simulink model "servo_armature"  (R2023b)
settings: Solver=ode45  StartTime=0.0  StopTime=Tend  MaxStep=1e-3  RelTol=1e-8  AbsTol=1e-10
model workspace (MAT data in the model file):
  J = 1e-06
  Kd = 0
  Ke = 0.00568713663315
  Ki = 1
  KiOn = 1
  Kp = 0.05
  Kt = 0.00568713663315
  L = 0.0005
  N = 100
  R = 1.6
  Tend = 5
  Tf = 0.01
  Ts = 0.01
  aw = 1
  b = 2.41369575255e-06
  closedLoop = 1
  dist = 0
  eta = 1
  ffGain = 0.0666666666667
  loopSel = 1
  qInt = 0.0692307692308
  setpoint = 100
  tDist = 3
  tStep = 0.2
  uMax = 12
libraries: simulink x2
settings Model: Creator=odyssix  LastModifiedBy=odyssix
settings ModelReferenceCC: UpdateModelReferenceTargets=IfOutOfDate
settings RTWCC: GPUComputeCapability=5.0
settings ConfigComp: CovBoundaryAbsTol=1.0e-5

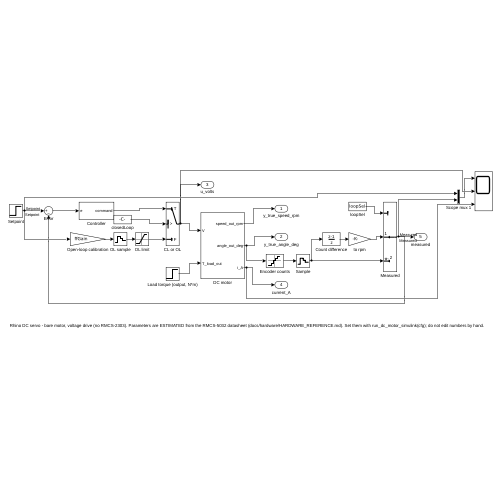
[thumbnail: Simulink's stored preview of the top-level diagram]
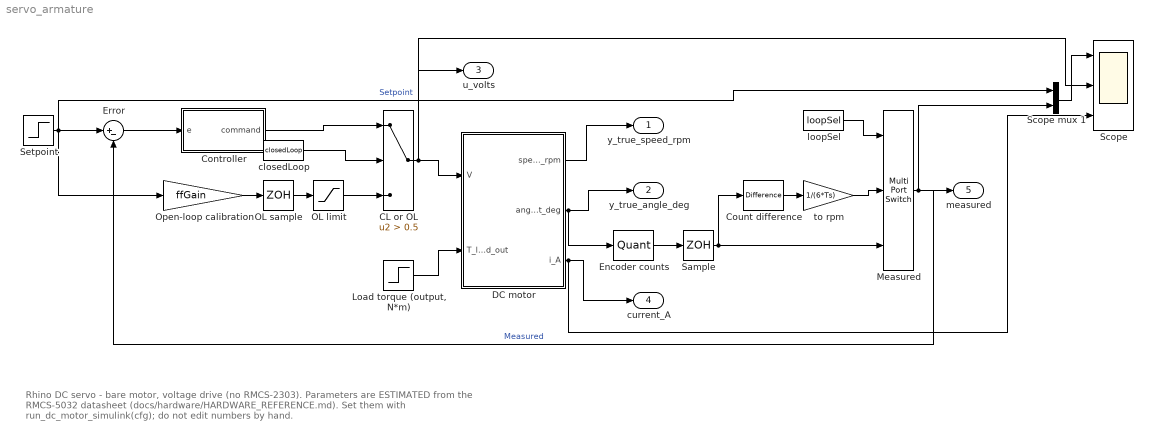
== system servo_armature ==
  note: Rhino DC servo - bare motor, voltage drive (no RMCS-2303). Parameters are ESTIMATED from the RMCS-5032 datasheet (docs/hardware/HARDWARE_REFERENCE.md). Set them with run_dc_motor_simulink(cfg); do not edit numbers by hand.
  CL or OL : Switch  Criteria=u2 > Threshold  Threshold=0.5  SaturateOnIntegerOverflow=off  InputSameDT=off
  Controller : Subsystem
  Count difference : simulink/Discrete/Difference  ICPrevInput=0.0  OutMin=[]  OutMax=[]  OutDataType=fixdt(1, 16)  OutScaling=2^-10  DoSatur=off
  DC motor : Subsystem
  Encoder counts : Quantizer  QuantizationInterval=qInt
  Error : Sum  Inputs=|+-
  "Load torque (output, N*m)" : Step  Time=tDist  After=dist  SampleTime=0
  Measured : MultiPortSwitch  Inputs=2  SaturateOnIntegerOverflow=off  InputSameDT=off
  OL limit : Saturate  UpperLimit=uMax  LowerLimit=-uMax
  OL sample : ZeroOrderHold  SampleTime=Ts
  Open-loop calibration : Gain  Gain=ffGain
  Sample : ZeroOrderHold  SampleTime=Ts
  Scope : Scope  NumInputPorts=3
  Scope mux 1 : Mux  Inputs=2
  Setpoint : Step  Time=tStep  After=setpoint  SampleTime=0
  closedLoop : Constant  Value=closedLoop
  loopSel : Constant  Value=loopSel
  to rpm : Gain  Gain=1/(6*Ts)
  y_true_speed_rpm : Outport
  y_true_angle_deg : Outport  Port=2
  u_volts : Outport  Port=3
  current_A : Outport  Port=4
  measured : Outport  Port=5
  wires:
  Setpoint/1 -> Error/1, Open-loop calibration/1, Scope mux 1/1  "Setpoint"
  Error/1 -> Controller/1(e)
  Controller/1(command) -> CL or OL/1
  closedLoop/1 -> CL or OL/2
  Open-loop calibration/1 -> OL sample/1
  OL sample/1 -> OL limit/1
  OL limit/1 -> CL or OL/3
  CL or OL/1 -> DC motor/1(V), u_volts/1, Scope/2
  "Load torque (output, N*m)"/1 -> DC motor/2(T_load_out)
  DC motor/1(speed_out_rpm) -> y_true_speed_rpm/1
  DC motor/2(angle_out_deg) -> y_true_angle_deg/1, Encoder counts/1
  DC motor/3(i_A) -> current_A/1, Scope/3
  Encoder counts/1 -> Sample/1
  Sample/1 -> Count difference/1, Measured/3
  Count difference/1 -> to rpm/1
  loopSel/1 -> Measured/1
  to rpm/1 -> Measured/2
  Measured/1 -> Error/2, measured/1, Scope mux 1/2  "Measured"
  Scope mux 1/1 -> Scope/1

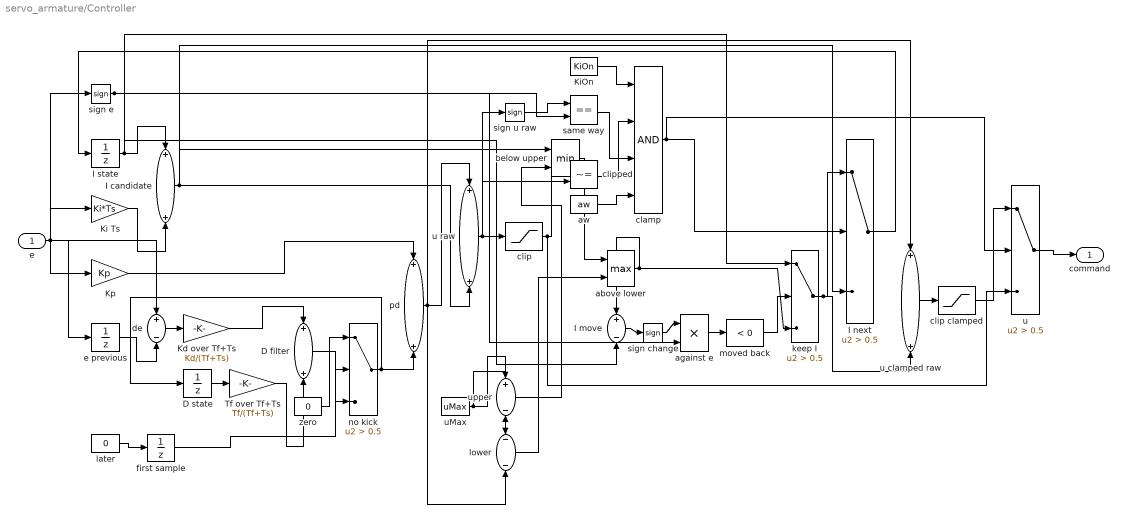
== system servo_armature/Controller ==
  e : Inport
  D filter : Sum
  D state : UnitDelay  SampleTime=Ts
  I candidate : Sum
  I move : Sum  Inputs=+-
  I next : Switch  Criteria=u2 > Threshold  Threshold=0.5  SaturateOnIntegerOverflow=off  InputSameDT=off
  I state : UnitDelay  SampleTime=Ts
  Kd over Tf+Ts : Gain  Gain=Kd/(Tf+Ts)
  Ki Ts : Gain  Gain=Ki*Ts
  KiOn : Constant  Value=KiOn
  Kp : Gain  Gain=Kp
  Tf over Tf+Ts : Gain  Gain=Tf/(Tf+Ts)
  above lower : MinMax  Function=max  Inputs=2
  against e : Product
  aw : Constant  Value=aw
  below upper : MinMax  Inputs=2
  clamp : Logic  Inputs=4  AllPortsSameDT=off  OutDataTypeStr=boolean
  clip : Saturate  UpperLimit=uMax  LowerLimit=-uMax
  clip clamped : Saturate  UpperLimit=uMax  LowerLimit=-uMax
  clipped : RelationalOperator  Operator=~=  OutDataTypeStr=boolean  RndMeth=Simplest  InputSameDT=off
  de : Sum  Inputs=+-
  e previous : UnitDelay  SampleTime=Ts
  first sample : UnitDelay  InitialCondition=1  SampleTime=Ts
  keep I : Switch  Criteria=u2 > Threshold  Threshold=0.5  SaturateOnIntegerOverflow=off  InputSameDT=off
  later : Constant  Value=0
  lower : Sum  Inputs=--
  moved back : simulink/Logic and Bit Operations/Compare To Constant  relop=<  const=0  OutDataTypeStr=boolean
  no kick : Switch  Criteria=u2 > Threshold  Threshold=0.5  SaturateOnIntegerOverflow=off  InputSameDT=off
  pd : Sum
  same way : RelationalOperator  Operator===  OutDataTypeStr=boolean  RndMeth=Simplest  InputSameDT=off
  sign change : Signum
  sign e : Signum
  sign u raw : Signum
  u : Switch  Criteria=u2 > Threshold  Threshold=0.5  SaturateOnIntegerOverflow=off  InputSameDT=off
  u clamped raw : Sum
  u raw : Sum
  uMax : Constant  Value=uMax
  upper : Sum  Inputs=+-
  zero : Constant  Value=0
  command : Outport
  wires:
  e/1 -> e previous/1, de/1, Ki Ts/1, Kp/1, sign e/1
  e previous/1 -> de/2
  de/1 -> Kd over Tf+Ts/1
  D state/1 -> Tf over Tf+Ts/1
  Kd over Tf+Ts/1 -> D filter/1
  Tf over Tf+Ts/1 -> D filter/2
  later/1 -> first sample/1
  zero/1 -> no kick/1
  first sample/1 -> no kick/2
  D filter/1 -> no kick/3
  no kick/1 -> D state/1, pd/2
  I state/1 -> I candidate/1, I move/2, keep I/1
  Ki Ts/1 -> I candidate/2
  Kp/1 -> pd/1
  pd/1 -> u raw/1, upper/2, lower/2, u clamped raw/1
  I candidate/1 -> u raw/2, below upper/1, I next/3
  u raw/1 -> clip/1, clipped/2, sign u raw/1
  clip/1 -> clipped/1, u/3
  sign u raw/1 -> same way/1
  sign e/1 -> same way/2, against e/2
  KiOn/1 -> clamp/1
  clipped/1 -> clamp/2
  same way/1 -> clamp/3
  aw/1 -> clamp/4
  uMax/1 -> upper/1, lower/1
  upper/1 -> below upper/2
  below upper/1 -> above lower/1
  lower/1 -> above lower/2
  above lower/1 -> I move/1, keep I/3
  I move/1 -> sign change/1
  sign change/1 -> against e/1
  against e/1 -> moved back/1
  moved back/1 -> keep I/2
  keep I/1 -> I next/1, u clamped raw/2
  clamp/1 -> I next/2, u/2
  I next/1 -> I state/1
  u clamped raw/1 -> clip clamped/1
  clip clamped/1 -> u/1
  u/1 -> command/1

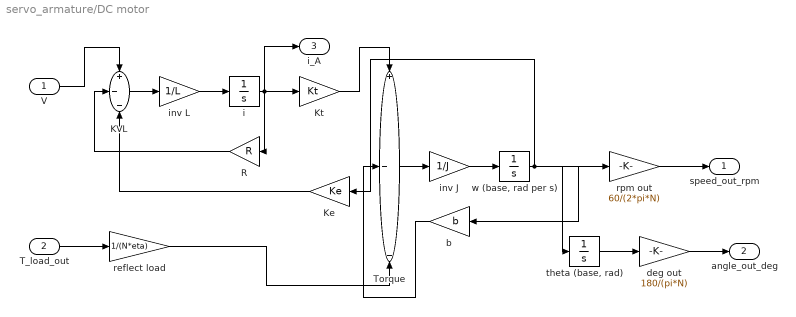
== system servo_armature/DC motor ==
  V : Inport
  T_load_out : Inport  Port=2
  KVL : Sum  Inputs=+--
  Ke : Gain  Gain=Ke
  Kt : Gain  Gain=Kt
  R : Gain  Gain=R
  Torque : Sum  Inputs=+--
  b : Gain  Gain=b
  deg out : Gain  Gain=180/(pi*N)
  i : Integrator
  inv J : Gain  Gain=1/J
  inv L : Gain  Gain=1/L
  reflect load : Gain  Gain=1/(N*eta)
  rpm out : Gain  Gain=60/(2*pi*N)
  "theta (base, rad)" : Integrator
  "w (base, rad per s)" : Integrator
  speed_out_rpm : Outport
  angle_out_deg : Outport  Port=2
  i_A : Outport  Port=3
  wires:
  V/1 -> KVL/1
  KVL/1 -> inv L/1
  inv L/1 -> i/1
  i/1 -> Kt/1, R/1, i_A/1
  R/1 -> KVL/2
  Kt/1 -> Torque/1
  Torque/1 -> inv J/1
  inv J/1 -> "w (base, rad per s)"/1
  "w (base, rad per s)"/1 -> b/1, Ke/1, "theta (base, rad)"/1, rpm out/1
  b/1 -> Torque/2
  Ke/1 -> KVL/3
  T_load_out/1 -> reflect load/1
  reflect load/1 -> Torque/3
  rpm out/1 -> speed_out_rpm/1
  "theta (base, rad)"/1 -> deg out/1
  deg out/1 -> angle_out_deg/1
